simulink model "Three_phase_line_fault_2018"  (R2018b)
settings: Solver=VariableStepAuto  StartTime=0.0  StopTime=0.04  FixedStep=1/2500  RelTol=1e-3
undefined symbols (not defined in the file or in its folder): D11, Delta
libraries: powerlib x10
settings Model: Creator=zyx  LastModifiedBy=zyx53
settings DebuggingCC: UnconnectedInputMsg=none  UnconnectedOutputMsg=none  UnconnectedLineMsg=none
settings ModelReferenceCC: EnableRefExpFcnMdlSchedulingChecks=off
settings RTWCC: Description=Generic Real-Time Target

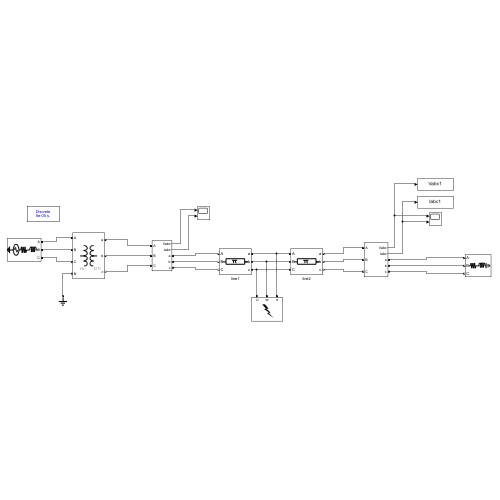
[thumbnail: Simulink's stored preview of the top-level diagram]
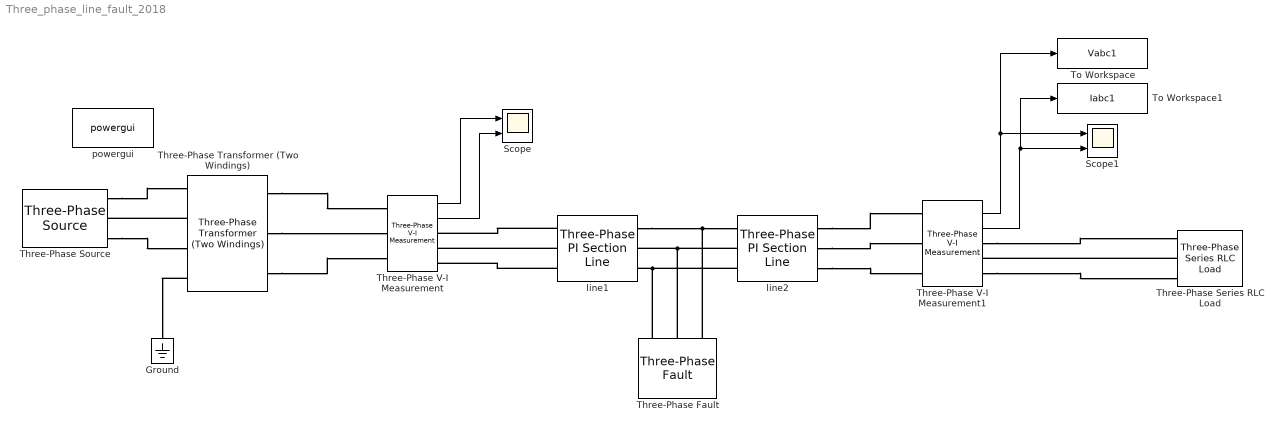
== system Three_phase_line_fault_2018 ==
  Ground : powerlib/Elements/Ground  LConnTagsString=a
  Scope : Scope  NumInputPorts=2
  Scope1 : Scope  NumInputPorts=2
  Three-Phase Series RLC Load : powerlib/Elements/Three-Phase Series RLC Load  LConnTagsString=A|B|C  Configuration=Y (grounded)  NominalVoltage=10.5e3  Vabc=[1e3 1e3 1e3]  Vabcp=[1e3 1e3 1e3]  NominalFrequency=50  UnbalancedPower=off  ActivePower=1.5e6  InductivePower=0.49e6  CapacitivePower=0  Pabc=[10e3 9e3 11e3]  QLabc=[100 90 110]  QCabc=[100 90 110]  Pabcp=[10e3 9e3 11e3]  QLabcp=[100 90 110]  QCabcp=[100 90 110]  Measurements=None  LoadType=constant Z
  Three-Phase Transformer (Two Windings) : powerlib/Elements/Three-Phase Transformer (Two Windings)  Winding1Connection=Yn  Winding2Connection=Delta (D11)  CoreType=Three single-phase transformers  SetSaturation=off  Hysteresis=off  DataFile='hysteresis'  SetInitialFlux=off  Measurements=None  UNITS=pu  NominalPower=[ 200e6 , 50 ]  Winding1=[ 110e3 , 0.002 , 0.08 ]  Winding2=[ 10.5e3 , 0.002 , 0.08 ]  Rm=500  Lm=500  L0=0.5  Saturation=[ 0,0 ; 0.0024,1.2 ; 1.0,1.52 ]  InitialFluxes=[ 0.8 , -0.8 , 0.7 ]  BreakLoop=off  DiscreteSolver=Trapezoidal iterative  DataType=off  TransfoNumber=1
  Three-Phase V-I Measurement : powerlib/Measurements/Three-Phase V-I Measurement  VoltageMeasurement=phase-to-ground  SetLabelV=off  LabelV=Vabc  Vpu=off  VpuLL=off  CurrentMeasurement=yes  SetLabelI=off  LabelI=Iabc  Ipu=off  Pbase=100e6  Vbase=500e3  OutputType=Complex  PhasorSimulation=off  PSBequivalent=0
  Three-Phase V-I Measurement1 : powerlib/Measurements/Three-Phase V-I Measurement  VoltageMeasurement=phase-to-ground  SetLabelV=off  LabelV=Vabc  Vpu=off  VpuLL=off  CurrentMeasurement=yes  SetLabelI=off  LabelI=Iabc  Ipu=off  Pbase=100e6  Vbase=500e3  OutputType=Complex  PhasorSimulation=off  PSBequivalent=0
  Three-Phase Fault : powerlib/Elements/Three-Phase Fault  InitialStates=0  FaultA=on  FaultB=off  FaultC=off  GroundFault=on  SwitchTimes=[0 ]  External=off  SwitchStatus=NaN  FaultResistance=0.001  GroundResistance=0.01  SnubberResistance=1e6  SnubberCapacitance=inf  Measurements=None
  Three-Phase Source : powerlib/Electrical Sources/Three-Phase Source  InternalConnection=Yg  VoltagePhases=off  Voltage=110e3  PhaseAngle=0  Voltage_phases=[25e3 25e3 25e3]/sqrt(3)  PhaseAngles_phases=[0 -120 +120]  Frequency=50  NonIdealSource=on  SpecifyImpedance=off  Resistance=5.74  Inductance=0.0452  ShortCircuitLevel=100e6  BaseVoltage=110e3/(3^0.5)  XRratio=7  BusType=swing  Pref=10e3  Qref=0  Prefabc=[10e3, 10e3, 10e3]  Qrefabc=[0, 0, 0]  Qmin=-inf  Qmax=inf
  To Workspace : ToWorkspace  VariableName=Vabc1  SaveFormat=Timeseries  SampleTime=0.0004
  To Workspace1 : ToWorkspace  VariableName=Iabc1  SaveFormat=Timeseries  SampleTime=0.0004
  line1 : powerlib/Elements/Three-Phase PI Section Line  LConnTagsString=a|b|c  RConnTagsString=A|B|C  Length=0.1  Frequency=60  Resistances=[ 0.01273 0.3864]  Inductances="[ 0.9337e-3  4.1264e-3]"  Capacitances=[12.74e-9 7.751e-9]
  line2 : powerlib/Elements/Three-Phase PI Section Line  LConnTagsString=a|b|c  RConnTagsString=A|B|C  Length=0.9  Frequency=60  Resistances=[ 0.01273 0.3864]  Inductances="[ 0.9337e-3  4.1264e-3]"  Capacitances=[12.74e-9 7.751e-9]
  powergui : powerlib/powergui  Priority=1  SimulationMode=Discrete  SampleTime=50e-6  frequency=60  Iterations=50  frequencyindice=50  Pbase=100e6  ErrMax=1e-4  UnitsV=kV  UnitsW=MW  buscounter=0  FunctionMessages=off  echomessages=off  EnableUseOfTLC=off  CurrentSourceSwitches=off  DisableSnubberDevices=off  DisableRonSwitches=off  DisableVfSwitches=off  DisplayEquations=off  AutomaticDiscreteSolvers=off  SolverType=Tustin/Backward Euler (TBE)  Interpol=off  ExternalGateDelay=off  methode=off  Ts=100  x0status=blocks  SPID=on  SwTol=0  HookPort=off  NonlinearTolerance=1e-4  nMaxIteration=100  ContinueOnMaxIteration=off  RestoreLinks=warning  ResistiveCurrentMeasurement=off  Frange=[0:2:500]  Ylog=off  Xlog=on  ShowGrid=off  save=off  variable=ZData  structure=0  ZoomFFT=off  StartTime=0.0  cycles=1  DisplayStyle=1  fundamental=60  FreqAxis=off  MaxFrequency=1000  frequencyindicesteady=1  RmsSteady=1  display=off
  wires:
  Three-Phase V-I Measurement/1 -> Scope/1
  Three-Phase V-I Measurement/2 -> Scope/2
  Three-Phase V-I Measurement1/1 -> To Workspace/1, Scope1/1
  Three-Phase V-I Measurement1/2 -> To Workspace1/1, Scope1/2
  connections:
  Three-Phase Series RLC Load/LConn2 -- Three-Phase V-I Measurement1/RConn2
  Three-Phase V-I Measurement1/RConn1 -- Three-Phase Series RLC Load/LConn1
  Three-Phase V-I Measurement1/RConn3 -- Three-Phase Series RLC Load/LConn3
  line1/LConn1 -- Three-Phase V-I Measurement/RConn1
  line1/LConn2 -- Three-Phase V-I Measurement/RConn2
  line1/LConn3 -- Three-Phase V-I Measurement/RConn3
  line1/RConn1 -- Three-Phase Fault/LConn1 -- line2/LConn1
  line2/LConn2 -- Three-Phase Fault/LConn2 -- line1/RConn2
  line2/LConn3 -- Three-Phase Fault/LConn3 -- line1/RConn3
  line2/RConn1 -- Three-Phase V-I Measurement1/LConn1
  line2/RConn2 -- Three-Phase V-I Measurement1/LConn2
  line2/RConn3 -- Three-Phase V-I Measurement1/LConn3
  Three-Phase Transformer (Two Windings)/LConn2 -- Three-Phase Source/RConn2
  Three-Phase Source/RConn1 -- Three-Phase Transformer (Two Windings)/LConn1
  Three-Phase Source/RConn3 -- Three-Phase Transformer (Two Windings)/LConn3
  Three-Phase Transformer (Two Windings)/LConn4 -- Ground/LConn1
  Three-Phase Transformer (Two Windings)/RConn1 -- Three-Phase V-I Measurement/LConn1
  Three-Phase Transformer (Two Windings)/RConn2 -- Three-Phase V-I Measurement/LConn2
  Three-Phase Transformer (Two Windings)/RConn3 -- Three-Phase V-I Measurement/LConn3
